simulink model "ELECTRIC_DRIVE"  (R2023a)
settings: Solver=ode1  StartTime=0.0  StopTime=tsim  FixedStep=CONTROL.Tm  RelTol=1e-3
undefined symbols (not defined in the file): CONTROL, MOTOR, myev, SENSOR, speed, tfalta, Tload, Vdc, VSC
libraries: simulink x9
(part 2 of 2)

== matlab function ELECTRIC_DRIVE/TORQUE CONTROL/Variant Subsystem/Vf_5Ph/Vf 5Phase PMSM ==
  settings: updateMethod=DISCRETE
  data: Vphase output; wm input; CONTROL parameter; Vdc parameter
function Vphase  = Vf_5PH(wm, CONTROL, Vdc)

% Variable init
persistent cntr;
persistent wm_km1;
persistent wt_km1;
persistent V_ph;

if isempty(cntr)
    cntr   = CONTROL.N_calc;
    wm_km1 = 0;
    wt_km1 = 0;
    V_ph   = zeros(5,1);
end


%---------  CONTROL LOOP  ---------%
if (cntr==CONTROL.N_calc)
    cntr=0;

    %----- VOLTAGE AMPLITUDE -----%
    Vn     = Vdc/2;
    V = Vn * wm/CONTROL.wm_n;

    %----- INTEGRATOR -----%
    wt = CONTROL.Ts*(wm + wm_km1)/2 + wt_km1;
    wm_km1 = wm;
    wt_km1 = wt;

    %----- VOLTAGE REFERENCE -----%
    ang    = 2*pi/CONTROL.Phase;
    V_ph(1,1) = V * cos(wt);
    V_ph(2,1) = V * cos(wt + ang);
    V_ph(3,1) = V * cos(wt + 2*ang);
    V_ph(4,1) = V * cos(wt + 3*ang);
    V_ph(5,1) = V * cos(wt + 4*ang);

end
cntr = cntr + 1;

%----- ACTUATION -----%
Vphase = V_ph;

end

== matlab function ELECTRIC_DRIVE/MOTOR/Variant Subsystem/PMSM_9Ph/ab2dq1 ==
  data: idq input; iab output; th input
function iab = Park(idq,th)

Mp= [ cos(th)  -sin(th)   0  0  0  0
      sin(th)   cos(th)   0  0  0  0
         0           0    1  0  0  0
         0           0    0  1  0  0
         0           0    0  0  1  0
         0           0    0  0  0  1];

iab = Mp*idq;
end

== matlab function ELECTRIC_DRIVE/TORQUE CONTROL/Variant Subsystem/MPC_9Ph_PMSM/MPC 9Phase PMSM ==
  settings: updateMethod=DISCRETE
  data: Iabc_med input; Sout output; vectores output; Tref input; wm input; th input; Fc_out output; IdqRef output; IabRef output; Iab_km1 output; ch output; CONTROL parameter; SENSOR parameter
function [Sout, vectores, Fc_out, IdqRef, IabRef, Iab_km1, ch] = FCS_MPC_9PH_PMSM(Iabc_med, Tref, wm, th, CONTROL, SENSOR)

% Variable init
persistent uk;
persistent cntr;
persistent x_opt;
% persistent Fc_ana;
persistent Fc;
persistent J_opt;
persistent dq_ref;
persistent Iab_ref;
persistent Sout_km1;
persistent cambios;
persistent Iabxy_med;
persistent Id_med;
persistent Iq_med;
persistent xkp1;
persistent Pkm1;

persistent th_km2;

persistent GAMMA;
persistent GAMMA_Vab;

if isempty(cntr)
    uk  = [0 0 0 0 0]';
    cntr= CONTROL.N_calc;
    Iab_ref = zeros(5,1);
    xkp1 = zeros(5,1);
    dq_ref = zeros(5,1);
    % Fc_ana = zeros(3*length(V_abxy) ,1);
    Fc     = 0;
    Sout_km1 = zeros(length(CONTROL.VECT.S(:,1)),1);
    Sout = zeros(length(CONTROL.VECT.S(:,1)),1);
    cambios = 0;
    x_opt = 0;
    Iabxy_med = zeros(CONTROL.Phase,1);
    Id_med = 0;
    Iq_med = 0;
    Pkm1 = zeros(5,5);

    th_km2 = th;

    GAMMA = CONTROL.B * CONTROL.Ts;
    GAMMA_Vab = GAMMA * CONTROL.Vdc*CONTROL.VECT.V_abxy;
end


%---------  CONTROL LOOP  ---------%
if (cntr==CONTROL.N_calc)
    cntr=0;

    we=wm*CONTROL.P;               % Electric speed
    th_km2 = th + 2*CONTROL.Ts*we; % Orientation correction

    % if MTPA == 1
    %     % v_max =  k_fw*Vdc/2;
    %     Is = sqrt(Id_ref^2 + Iq_ref^2);
    %     kfilt = 0.4;
    %     Iq_med_filt = kfilt*Iq_med + (1-kfilt)*Iq_med_filt;
    %     Id_med_filt = kfilt*Id_med + (1-kfilt)*Id_med_filt;
    % 
    %     Cond_1 = (v_max/we)^2;
    %     Cond_2 = (EMcontrolMPC.Lq*Iq_med_filt)^2+(EMcontrolMPC.Ld*Id_med_filt+EMcontrolMPC.Lambda)^2;
    % 
    %     if 0.8* Cond_1 > Cond_2   % Para evitar singularidades de las referencias de FW
    %         Id_ref = (-EMcontrolMPC.Lambda+sqrt(EMcontrolMPC.Lambda^2 + 8*((EMcontrolMPC.Ld-EMcontrolMPC.Lq)^2)*Is^2)) / (4*(EMcontrolMPC.Ld-EMcontrolMPC.Lq));
    %         Iq_ref = (2*Te_ref) / ( 9*EMcontrolMPC.P * (EMcontrolMPC.Lambda+(EMcontrolMPC.Ld-EMcontrolMPC.Lq)*Id_ref) );
    %     else
    %         Id_ref_mtpa = (-EMcontrolMPC.Lambda+sqrt(EMcontrolMPC.Lambda^2 + 8*((EMcontrolMPC.Ld-EMcontrolMPC.Lq)^2)*Is^2)) / (4*(EMcontrolMPC.Ld-EMcontrolMPC.Lq));
    %         Iq_ref_mtpa = (2*Te_ref) / ( 9*EMcontrolMPC.P * (EMcontrolMPC.Lambda+(EMcontrolMPC.Ld-EMcontrolMPC.Lq)*Id_ref_mtpa) );
    % 
    %         arg = (EMcontrolMPC.Lambda * EMcontrolMPC.Ld)^2 - (EMcontrolMPC.Ld^2 - EMcontrolMPC.Lq^2) * (EMcontrolMPC.Lambda + (EMcontrolMPC.Lq^2) * Is^2 - (v_max^2) / we^2);
    %         if arg > 0 % Control del argumento de la raiz
    %             Id_ref_fw   = (-EMcontrolMPC.Lambda * EMcontrolMPC.Ld + sqrt( arg )) / (EMcontrolMPC.Ld^2 - EMcontrolMPC.Lq^2);
    %             Iq_ref_fw   = (2*Te_ref) / ( 9*EMcontrolMPC.P * (EMcontrolMPC.Lambda+(EMcontrolMPC.Ld-EMcontrolMPC.Lq)*Id_ref_fw) );
    %             beta_mtpa = atan2(Iq_ref_mtpa, Id_ref_mtpa);
    %             beta_fw   = atan2(Iq_ref_fw  , Id_ref_fw  );
    % 
    %             if beta_fw < beta_mtpa   % Zona MTPA
    %                 Id_ref = Id_ref_mtpa;
    %                 Iq_ref = Iq_ref_mtpa;
    % 
    %             else % Zona Field Weakening
    %                 Id_ref = Id_ref_fw;
    %                 Iq_ref = Iq_ref_fw;
    %             end
    %         else
    %             Id_ref = Id_ref_mtpa;
    %             Iq_ref = Iq_ref_mtpa;
    %         end
    %     end
    % else
    % Iq_ref = (2/9)*Te_ref / (EMcontrolMPC.P*EMcontrolMPC.Lambda);
    % end

    %----- REFERENCE CURRENTS -----%
    Id_ref  = 0;
    Iq_ref  = (2/CONTROL.Phase) * Tref/(CONTROL.P*CONTROL.Lambda); 
    Id2_ref = 0;
    Iq2_ref = 0;
    Id3_ref = 0;
    Iq3_ref = 0;
    Ih_ref  = 0;

    % Saturation
    if (Iq_ref >= CONTROL.In)
        Iq_ref = CONTROL.In;
    elseif (Iq_ref <= -CONTROL.In)
        Iq_ref = -CONTROL.In;
    end

    % Inverse Park transform
    Ia_ref = Id_ref*cos(th_km2)    - Iq_ref*sin(th_km2);
    Ib_ref = Id_ref*sin(th_km2)    + Iq_ref*cos(th_km2);
    Ix1_ref = 0; % Id2_ref*cos(3*th_km2) - Iq2_ref*sin(3*th_km2);
    Iy1_ref = 0; % Id2_ref*sin(3*th_km2) + Iq2_ref*cos(3*th_km2);
    Ix2_ref = 0; % Id2_ref*cos(3*th_km2) - Iq2_ref*sin(3*th_km2);
    Iy2_ref = 0; % Id2_ref*sin(3*th_km2) + Iq2_ref*cos(3*th_km2);

    dq_ref  = [Id_ref Iq_ref  Id2_ref Iq2_ref  Id3_ref Iq3_ref  Ih_ref]';
    Iab_ref = [Ia_ref Ib_ref  Ix1_ref Iy1_ref  Ix2_ref Iy2_ref  Ih_ref]';

    %-----   STATE SPACE   -----%
    Ap=[ 0    (CONTROL.Lq*we)/CONTROL.Ld  0    0    0    0
    (CONTROL.Ld*we)/CONTROL.Lq  0         0    0    0    0
         0                      0         0    0    0    0
         0                      0         0    0    0    0
         0                      0         0    0    0    0
         0                      0         0    0    0    0];
    FI=(eye(CONTROL.Phase) + (CONTROL.A+Ap) *CONTROL.Ts); % Discrete state space

    Bemf = [0 -(lambda*we)/Lq 0 0 0 0]';

    %-----  CURRENT MEASUREMENT  -----%
    Iph_sensor = Iabc_med + SENSOR.CURRENT.sigma*randn(9,1);
    
    %  Filtro de Kalman 
    if CONTROL.KALMAN.ACTIVE == 1
        Iph_k = CONTROL.invClarke * xkp1;
        Pk = FI*Pkm1*inv(FI) + CONTROL.KALMAN.Q;
        kk = Pk*inv(Pk + CONTROL.KALMAN.R);
        Iph_filt = Iph_k + kk*(Iph_sensor - Iph_k);
        Pkm1 = (eye(5)-kk)*Pk;
    else
        Iph_filt = Iph_sensor;
    end

    Iabxy_med = CONTROL.Clarke*Iph_filt;
    Id_med =  Iabxy_med(1)*cos(th) + Iabxy_med(2)*sin(th); %Transformada de Park sincrona
    Iq_med = -Iabxy_med(1)*sin(th) + Iabxy_med(2)*cos(th);
    xk = [Id_med Iq_med Iabxy_med(3) Iabxy_med(4) Iabxy_med(5)  Iabxy_med(6) Iabxy_med(7) Iabxy_med(8) Iabxy_med(9)]';

    %----- PREDICTION k+1 -----%
    xkp1=FI*xk + GAMMA*(uk + Bemf);

    %----- PREDICTION k+2 (CONSTANT) -----%
    xkp2_cnst = FI*xkp1 + Bemf*CONTROL.Ts;

    %---- OPTIMIZATION LOOP - PREDICTION k+2 ----%
    Mp= [ cos(th) sin(th) 0  0  0  0 
         -sin(th) cos(th) 0  0  0  0
           0       0      1  0  0  0
           0       0      0  1  0  0
           0       0      0  0  1  0
           0       0      0  0  0  1];

    GAMMA_Vdq = Mp*GAMMA_Vab(1:6,:);
    J_opt = inf; %Inicializacion de la funcion de coste
    for m=1:length(CONTROL.VECT.indx)
        xkp2  = xkp2_cnst + GAMMA_Vdq(:,CONTROL.VECT.indx(m));% xkp2  = FI*xkp1 + GAMMA*V_abxy(:,m) + DELTA;
        error = dq_ref - xkp2;

        Fc1 = error(1)^2 + CONTROL.Kd*error(2)^2;
        Fc2 = CONTROL.Kx1*error(3)^2 + CONTROL.Ky1*error(4)^2;
        Fc3 = CONTROL.Kx2*error(5)^2 + CONTROL.Ky2*error(6)^2;
        %Fc3 = CONTROL.Kh*(error(5)^2);    % Fc_ana(m) = Fc1; Fc_ana(m + length(V_abxy)) = Fc2; Fc_ana(m + 2*length(V_abxy)) = Fc3;

        Fc = Fc1 + Fc2 + Fc3;

        if (Fc < J_opt)
            J_opt=Fc;
            x_opt = m;
        end
    end
    % Voltage vector update
    uk = CONTROL.Vdc* Mp * CONTROL.VECT.V_abxy(:,CONTROL.VECT.indx(x_opt));

    % Swith_km2ing frec. calculation
    cambios = cambios + sum(abs(CONTROL.VECT.S(:,CONTROL.VECT.indx(x_opt)) - Sout_km1)); 
    Sout_km1 = CONTROL.VECT.S(:,CONTROL.VECT.indx(x_opt));
end
cntr = cntr + 1;

%----- ACTUATION -----%
Sout = Sout_km1;

% Output Variable Update
IdqRef = dq_ref;
IabRef = Iab_ref;
Iab_km1 = xkp1;
Fc_out = Fc;
vectores = CONTROL.VECT.indx(x_opt);
ch = cambios;
end

== matlab function ELECTRIC_DRIVE/MOTOR/Variant Subsystem/IM_6Ph/ab2dq ==
  data: Vabxy input; Vdqxy output; th input
 function Vdqxy = Park(Vabxy,th)

% Mp= [ cos(th)   sin(th)           0         0          0
%      -sin(th)   cos(th)           0         0          0 
%          0           0        cos(3*th)   -sin(3*th)   0
%          0           0        sin(3*th)    cos(3*th)   0
%          0           0            0         0          1];
Vdqxy = zeros(5,1);
Mp= [ cos(th)   sin(th)  0  0  0
     -sin(th)   cos(th)  0  0  0 
         0           0   1  0  0
         0           0   0  1  0
         0           0   0  0  1];

Vdqxy = Mp*Vabxy;
end

== matlab function ELECTRIC_DRIVE/TORQUE CONTROL/Variant Subsystem/FOC_5Ph/FOC 5Phase PMSM ==
  settings: updateMethod=DISCRETE
  data: Iabc_med input; Vph_ref output; Tref input; wm input; th input; IdqRef output; IabRef output; CONTROL parameter; SENSOR parameter; VdqRef output; VabRef output
function [Vph_ref, IdqRef, IabRef, VdqRef, VabRef] = FOC_5PH_PMSM(Iabc_med, Tref, wm, th, CONTROL, SENSOR)

% Variable init
persistent cntr;
persistent Vabc_ref;
persistent dq_ref;
persistent Iab_ref;
persistent Iabxy_med;
persistent Vdqxy_ref Vabxy;
persistent Pkm1;

persistent iderror_km1 idinte_km1 iqerror_km1 iqinte_km1;
persistent id3error_km1 id3inte_km1 iq3error_km1 iq3inte_km1 iherror_km1 ihinte_km1;

if isempty(cntr)
    Vabc_ref  = zeros(5,1);%[0 0 0 0 0]';
    cntr= CONTROL.N_calc;
    Iab_ref = zeros(5,1);
    dq_ref = zeros(5,1);
    Iabxy_med = zeros(CONTROL.Phase,1);
    Vdqxy_ref = zeros(5,1); Vabxy = zeros(5,1);
    iderror_km1 = 0; idinte_km1 = 0; iqerror_km1 = 0; iqinte_km1 = 0;
    id3error_km1 = 0; id3inte_km1 = 0; iq3error_km1 = 0; iq3inte_km1 = 0; iherror_km1 = 0; ihinte_km1 = 0;
    Pkm1 = zeros(5,5);
end


%---------  CONTROL LOOP  ---------%
if (cntr==CONTROL.N_calc)
    cntr=0;

    %------- REFERENCE CURRENTS -------%
    Id_ref  = 0;
    Iq_ref  = (2/CONTROL.Phase) * Tref/(CONTROL.P*CONTROL.Lambda); 
    Id3_ref = 0;
    Iq3_ref = 0;
    Ih_ref  = 0;

    % Saturation
    if (Iq_ref >= CONTROL.In)
        Iq_ref = CONTROL.In;
    elseif (Iq_ref <= -CONTROL.In)
        Iq_ref = -CONTROL.In;
    end

    % Inverse Park transform
    Ia_ref = Id_ref*cos(th)    - Iq_ref*sin(th);
    Ib_ref = Id_ref*sin(th)    + Iq_ref*cos(th);
    Ix_ref = Id3_ref*cos(3*th) - Iq3_ref*sin(3*th);
    Iy_ref = Id3_ref*sin(3*th) + Iq3_ref*cos(3*th);

    dq_ref  = [Id_ref Iq_ref Id3_ref Iq3_ref Ih_ref]';
    Iab_ref = [Ia_ref Ib_ref Ix_ref  Iy_ref  Ih_ref]';


    %-------  CURRENT MEASUREMENT  -------%
    % Iph_sensor = Iabc_med + SENSOR.CURRENT.sigma*randn(5,1);
    % 
    % %  Filtro de Kalman 
    % if CONTROL.KALMAN.ACTIVE == 1
    %     Iph_k = CONTROL.invClarke * xkp1;
    %     Pk = FI*Pkm1*inv(FI) + CONTROL.KALMAN.Q;
    %     kk = Pk*inv(Pk + CONTROL.KALMAN.R);
    %     Iph_filt = Iph_k + kk*(Iph_sensor - Iph_k);
    %     Pkm1 = (eye(5)-kk)*Pk;
    % else
    %     Iph_filt = Iph_sensor;
    % end
    Iph_filt = Iabc_med;

    Iabxy_med = CONTROL.Clarke*Iph_filt;

    Id_mea  =  Iabxy_med(1)*cos(th)   + Iabxy_med(2)*sin(th);
    Iq_mea  = -Iabxy_med(1)*sin(th)   + Iabxy_med(2)*cos(th);
    Id3_mea =  Iabxy_med(3)*cos(3*th) + Iabxy_med(4)*sin(3*th); 
    Iq3_mea = -Iabxy_med(3)*sin(3*th) + Iabxy_med(4)*cos(3*th);
    Ih_mea  =  Iabxy_med(5);


    %------------------ PI: D Voltage ------------------%
    id_error=Id_ref-Id_mea; 
    idinte_k = 0.5*CONTROL.Ts*(id_error+iderror_km1)+idinte_km1;
    Vd_ref = CONTROL.id.Kp*id_error + CONTROL.id.Ki*idinte_k;

        % Update variables
        iderror_km1 = id_error;
        idinte_km1  = idinte_k;

    %------------------ PI: Q Voltage ------------------%
    iq_error=Iq_ref-Iq_mea; 
    iqinte_k = 0.5*CONTROL.Ts*(iq_error+iqerror_km1)+iqinte_km1;
    Vq_ref = CONTROL.iq.Kp*iq_error + CONTROL.iq.Ki*iqinte_k;

        % Update variables
        iqerror_km1 = iq_error;
        iqinte_km1  = iqinte_k;

    %------------------ PI: D3 Voltage ------------------%
    id3_error=Id3_ref-Id3_mea; 
    id3inte_k = 0.5*CONTROL.Ts*(id3_error+id3error_km1)+id3inte_km1;
    Vd3_ref = CONTROL.id3.Kp*id3_error + CONTROL.id3.Ki*id3inte_k;

        % Update variables
        id3error_km1 = id3_error;
        id3inte_km1  = id3inte_k;

    %------------------ PI: Q3 Voltage ------------------%
    iq3_error=Iq3_ref-Iq3_mea; 
    iq3inte_k = 0.5*CONTROL.Ts*(iq3_error+iq3error_km1)+iq3inte_km1;
    Vq3_ref = CONTROL.iq3.Kp*iq3_error + CONTROL.iq3.Ki*iq3inte_k;

        % Update variables
        iq3error_km1 = iq3_error;
        iq3inte_km1  = iq3inte_k;

    %------------- PI: zero-sequence Voltage -------------%
    ih_error=Ih_ref-Ih_mea;
    ihinte_k = 0.5*CONTROL.Ts*(ih_error+iherror_km1)+ihinte_km1;
    Vh_ref = CONTROL.ih.Kp*ih_error + CONTROL.ih.Ki*ihinte_k;

        % Update variables
        iherror_km1 = ih_error;
        ihinte_km1  = ihinte_k;


    %-------  REFERENCE VOLTAGE TRANSFORMATIONS  -------%
    Vdqxy_ref = [Vd_ref; Vq_ref; Vd3_ref; Vq3_ref; Vh_ref];

    % Alpha-beta voltage
    Valpha_ref =  Vd_ref*cos(th)  - Vq_ref*sin(th); %Transformada de Park sincrona
    Vbeta_ref  =  Vd_ref*sin(th)  + Vq_ref*cos(th);
    Vx_ref   =  Vd3_ref*cos(3*th) - Vq3_ref*sin(3*th); %Transformada de Park anti-sincrona
    Vy_ref   =  Vd3_ref*sin(3*th) + Vq3_ref*cos(3*th);

    Vabxy = [Valpha_ref; Vbeta_ref; Vx_ref; Vy_ref; Vh_ref];

    % Phase voltage
    Vabc_ref = CONTROL.invClarke*Vabxy;
end
cntr = cntr + 1;

%----- ACTUATION -----%
Vph_ref = Vabc_ref;

% Output Variable Update
IdqRef = dq_ref;
IabRef = Iab_ref;
VdqRef = Vdqxy_ref;
VabRef = Vabxy;
end

== matlab function ELECTRIC_DRIVE/TORQUE CONTROL/Variant Subsystem/FOC_5Ph/MODULATION STAGE/DutyCicle ==
  data: dph input; dl output
function dl = fcn(dph)

dl = zeros(10,1);

if dph(1)>0
    dl(1) = dph(1);
else
    dl(6) = -1*dph(1);
end

if dph(2)>0
    dl(2) = dph(2);
else
    dl(7) = -1*dph(2);
end

if dph(3)>0
    dl(3) = dph(3);
else
    dl(8) = -1*dph(3);
end

if dph(4)>0
    dl(4) = dph(4);
else
    dl(9) = -1*dph(4);
end

if dph(5)>0
    dl(5) = dph(5);
else
    dl(10) = -1*dph(5);
end

== matlab function ELECTRIC_DRIVE/TORQUE CONTROL/Output select ==
  data: o4 input; vect output; o5 input; o6 input; ch output; Iabkm1 output; Vdq_ref output; Vab_ref output; CONTROL parameter
function [vect, ch, Iabkm1, Vdq_ref, Vab_ref]   = output(o4,o5,o6, CONTROL)

vect = 0;
ch = 0;
Iabkm1 = zeros(CONTROL.Phase,1);    
Vdq_ref = zeros(CONTROL.Phase,1);
Vab_ref = zeros(CONTROL.Phase,1);

if CONTROL.Index == 51 || CONTROL.Index == 91  % MPC
    vect = o4;
    ch   = o5;
    Iabkm1 = o6;
elseif CONTROL.Index == 52 || CONTROL.Index == 92 % FOC 
    Vdq_ref = o4;
    Vab_ref = o5;
end

end

== matlab function ELECTRIC_DRIVE/TORQUE CONTROL/Variant Subsystem/FOC_6Ph/FOC 6Phase PMSM ==
  settings: updateMethod=DISCRETE
  data: Iabc_med input; Vph_ref output; Tref input; wm input; th input; IdqRef output; IabRef output; CONTROL parameter; SENSOR parameter; VdqRef output; VabRef output
function [Vph_ref, IdqRef, IabRef, VdqRef, VabRef] = FOC_6PH(Iabc_med, Tref, wm, th, CONTROL, SENSOR)

% Variable init
persistent cntr;
persistent Vabc_ref;
persistent dq_ref;
persistent Iab_ref;
persistent Iabxy_med;
persistent Vdqxy_ref Vabxy;
persistent Pkm1;

persistent iderror_km1 idinte_km1 iqerror_km1 iqinte_km1;
persistent id3error_km1 id3inte_km1 iq3error_km1 iq3inte_km1 iherror_km1 ihinte_km1;

if isempty(cntr)
    Vabc_ref  = zeros(5,1);%[0 0 0 0 0]';
    cntr= CONTROL.N_calc;
    Iab_ref = zeros(5,1);
    dq_ref = zeros(5,1);
    Iabxy_med = zeros(CONTROL.Phase,1);
    Vdqxy_ref = zeros(5,1); Vabxy = zeros(5,1);
    iderror_km1 = 0; idinte_km1 = 0; iqerror_km1 = 0; iqinte_km1 = 0;
    id3error_km1 = 0; id3inte_km1 = 0; iq3error_km1 = 0; iq3inte_km1 = 0; iherror_km1 = 0; ihinte_km1 = 0;
    Pkm1 = zeros(5,5);
end


%---------  CONTROL LOOP  ---------%
if (cntr==CONTROL.N_calc)
    cntr=0;

    %------- REFERENCE CURRENTS -------%
    Id_ref  = 0;
    Iq_ref  = (2/CONTROL.Phase) * Tref/(CONTROL.P*CONTROL.Lambda); 
    Id5_ref = 0;
    Iq5_ref = 0;

    % Saturation
    if (Iq_ref >= CONTROL.In)
        Iq_ref = CONTROL.In;
    elseif (Iq_ref <= -CONTROL.In)
        Iq_ref = -CONTROL.In;
    end

    % Inverse Park transform
    Ia_ref = Id_ref*cos(th)    - Iq_ref*sin(th);
    Ib_ref = Id_ref*sin(th)    + Iq_ref*cos(th);
    Ix_ref = Id3_ref*cos(3*th) - Iq3_ref*sin(3*th);
    Iy_ref = Id3_ref*sin(3*th) + Iq3_ref*cos(3*th);

    dq_ref  = [Id_ref Iq_ref Id3_ref Iq3_ref Ih_ref]';
    Iab_ref = [Ia_ref Ib_ref Ix_ref  Iy_ref  Ih_ref]';


    %-------  CURRENT MEASUREMENT  -------%
    % Iph_sensor = Iabc_med + SENSOR.CURRENT.sigma*randn(5,1);
    % 
    % %  Filtro de Kalman 
    % if CONTROL.KALMAN.ACTIVE == 1
    %     Iph_k = CONTROL.invClarke * xkp1;
    %     Pk = FI*Pkm1*inv(FI) + CONTROL.KALMAN.Q;
    %     kk = Pk*inv(Pk + CONTROL.KALMAN.R);
    %     Iph_filt = Iph_k + kk*(Iph_sensor - Iph_k);
    %     Pkm1 = (eye(5)-kk)*Pk;
    % else
    %     Iph_filt = Iph_sensor;
    % end
    Iph_filt = Iabc_med;

    Iabxy_med = CONTROL.Clarke*Iph_filt;

    Id_mea  =  Iabxy_med(1)*cos(th)   + Iabxy_med(2)*sin(th);
    Iq_mea  = -Iabxy_med(1)*sin(th)   + Iabxy_med(2)*cos(th);
    Id3_mea =  Iabxy_med(3)*cos(3*th) + Iabxy_med(4)*sin(3*th); 
    Iq3_mea = -Iabxy_med(3)*sin(3*th) + Iabxy_med(4)*cos(3*th);
    Ih_mea  =  Iabxy_med(5);


    %------------------ PI: D Voltage ------------------%
    id_error=Id_ref-Id_mea; 
    idinte_k = 0.5*CONTROL.Ts*(id_error+iderror_km1)+idinte_km1;
    Vd_ref = CONTROL.id.Kp*id_error + CONTROL.id.Ki*idinte_k;

        % Update variables
        iderror_km1 = id_error;
        idinte_km1  = idinte_k;

    %------------------ PI: Q Voltage ------------------%
    iq_error=Iq_ref-Iq_mea; 
    iqinte_k = 0.5*CONTROL.Ts*(iq_error+iqerror_km1)+iqinte_km1;
    Vq_ref = CONTROL.iq.Kp*iq_error + CONTROL.iq.Ki*iqinte_k;

        % Update variables
        iqerror_km1 = iq_error;
        iqinte_km1  = iqinte_k;

    %------------------ PI: D3 Voltage ------------------%
    id3_error=Id3_ref-Id3_mea; 
    id3inte_k = 0.5*CONTROL.Ts*(id3_error+id3error_km1)+id3inte_km1;
    Vd3_ref = CONTROL.id3.Kp*id3_error + CONTROL.id3.Ki*id3inte_k;

        % Update variables
        id3error_km1 = id3_error;
        id3inte_km1  = id3inte_k;

    %------------------ PI: Q3 Voltage ------------------%
    iq3_error=Iq3_ref-Iq3_mea; 
    iq3inte_k = 0.5*CONTROL.Ts*(iq3_error+iq3error_km1)+iq3inte_km1;
    Vq3_ref = CONTROL.iq3.Kp*iq3_error + CONTROL.iq3.Ki*iq3inte_k;

        % Update variables
        iq3error_km1 = iq3_error;
        iq3inte_km1  = iq3inte_k;

    %------------- PI: zero-sequence Voltage -------------%
    ih_error=Ih_ref-Ih_mea;
    ihinte_k = 0.5*CONTROL.Ts*(ih_error+iherror_km1)+ihinte_km1;
    Vh_ref = CONTROL.ih.Kp*ih_error + CONTROL.ih.Ki*ihinte_k;

        % Update variables
        iherror_km1 = ih_error;
        ihinte_km1  = ihinte_k;


    %-------  REFERENCE VOLTAGE TRANSFORMATIONS  -------%
    Vdqxy_ref = [Vd_ref; Vq_ref; Vd3_ref; Vq3_ref; Vh_ref];

    % Alpha-beta voltage
    Valpha_ref =  Vd_ref*cos(th)  - Vq_ref*sin(th); %Transformada de Park sincrona
    Vbeta_ref  =  Vd_ref*sin(th)  + Vq_ref*cos(th);
    Vx_ref   =  Vd3_ref*cos(3*th) - Vq3_ref*sin(3*th); %Transformada de Park anti-sincrona
    Vy_ref   =  Vd3_ref*sin(3*th) + Vq3_ref*cos(3*th);

    Vabxy = [Valpha_ref; Vbeta_ref; Vx_ref; Vy_ref; Vh_ref];

    % Phase voltage
    Vabc_ref = CONTROL.invClarke*Vabxy;
end
cntr = cntr + 1;

%----- ACTUATION -----%
Vph_ref = Vabc_ref;

% Output Variable Update
IdqRef = dq_ref;
IabRef = Iab_ref;
VdqRef = Vdqxy_ref;
VabRef = Vabxy;
end

== matlab function ELECTRIC_DRIVE/TORQUE CONTROL/Variant Subsystem/FOC_6Ph/MODULATION STAGE/DutyCicle ==
  data: dph input; dl output
function dl = fcn(dph)

dl = zeros(10,1);

if dph(1)>0
    dl(1) = dph(1);
else
    dl(6) = -1*dph(1);
end

if dph(2)>0
    dl(2) = dph(2);
else
    dl(7) = -1*dph(2);
end

if dph(3)>0
    dl(3) = dph(3);
else
    dl(8) = -1*dph(3);
end

if dph(4)>0
    dl(4) = dph(4);
else
    dl(9) = -1*dph(4);
end

if dph(5)>0
    dl(5) = dph(5);
else
    dl(10) = -1*dph(5);
end

== matlab function ELECTRIC_DRIVE/MOTOR/Variant Subsystem/PMSM_9Ph/ab2dq ==
  data: Vabxy input; Vdqxy output; th input
function Vdqxy = Park(Vabxy,th)

Mp= [ cos(th)   sin(th)   0  0  0  0
     -sin(th)   cos(th)   0  0  0  0
         0           0    1  0  0  0
         0           0    0  1  0  0
         0           0    0  0  1  0
         0           0    0  0  0  1];

Vdqxy = Mp*Vabxy;
end

== matlab function ELECTRIC_DRIVE/TORQUE CONTROL/Variant Subsystem/Hybrid_PI&MPC/Hybrid PIdq and MPCh 5Ph ==
  settings: updateMethod=DISCRETE
  data: Iabc_med input; Vph_ref output; Tref input; wm input; th input; IdqRef output; IabRef output; CONTROL parameter; SENSOR parameter; VdqRef output; VabRef output
function [Vph_ref, IdqRef, IabRef, VdqRef, VabRef] = Hybrid_PIMPC(Iabc_med, Tref, wm, th, CONTROL, SENSOR)

% Variable init
persistent cntr;
persistent Vabc_ref;
persistent dq_ref;
persistent Iab_ref;
persistent Iabxy_med;
persistent Vdqxy_ref Vabxy;
persistent Pkm1;

persistent iderror_km1 idinte_km1 iqerror_km1 iqinte_km1;
persistent id3error_km1 id3inte_km1 iq3error_km1 iq3inte_km1 iherror_km1 ihinte_km1;

persistent FIh GAMMAh uh_k;

if isempty(cntr)
    Vabc_ref  = zeros(5,1);%[0 0 0 0 0]';
    cntr= CONTROL.N_calc;
    Iab_ref = zeros(5,1);
    dq_ref = zeros(5,1);
    Iabxy_med = zeros(CONTROL.Phase,1);
    Vdqxy_ref = zeros(5,1); Vabxy = zeros(5,1);
    iderror_km1 = 0; idinte_km1 = 0; iqerror_km1 = 0; iqinte_km1 = 0;
    id3error_km1 = 0; id3inte_km1 = 0; iq3error_km1 = 0; iq3inte_km1 = 0; iherror_km1 = 0; ihinte_km1 = 0;
    Pkm1 = zeros(5,5);

    uh_k = 0;
    FIh    = (1 + CONTROL.Ah*CONTROL.Ts);
    GAMMAh = CONTROL.Bh * CONTROL.Ts;
end


%---------  CONTROL LOOP  ---------%
if (cntr==CONTROL.N_calc)
    cntr=0;
    we = wm*CONTROL.P;

    %------- REFERENCE CURRENTS -------%
    Id_ref  = 0;
    Iq_ref  = (2/CONTROL.Phase) * Tref/(CONTROL.P*CONTROL.Lambda); 
    Id3_ref = 0;
    Iq3_ref = 0;
    Ih_ref  = 0;

    % Saturation
    if (Iq_ref >= CONTROL.In)
        Iq_ref = CONTROL.In;
    elseif (Iq_ref <= -CONTROL.In)
        Iq_ref = -CONTROL.In;
    end

    % Inverse Park transform
    Ia_ref = Id_ref*cos(th)    - Iq_ref*sin(th);
    Ib_ref = Id_ref*sin(th)    + Iq_ref*cos(th);
    Ix_ref = Id3_ref*cos(3*th) - Iq3_ref*sin(3*th);
    Iy_ref = Id3_ref*sin(3*th) + Iq3_ref*cos(3*th);

    dq_ref  = [Id_ref Iq_ref Id3_ref Iq3_ref Ih_ref]';
    Iab_ref = [Ia_ref Ib_ref Ix_ref  Iy_ref  Ih_ref]';


    %-------  CURRENT MEASUREMENT  -------%
    % Iph_sensor = Iabc_med + SENSOR.CURRENT.sigma*randn(5,1);
    % 
    % %  Filtro de Kalman 
    % if CONTROL.KALMAN.ACTIVE == 1
    %     Iph_k = CONTROL.invClarke * xkp1;
    %     Pk = FI*Pkm1*inv(FI) + CONTROL.KALMAN.Q;
    %     kk = Pk*inv(Pk + CONTROL.KALMAN.R);
    %     Iph_filt = Iph_k + kk*(Iph_sensor - Iph_k);
    %     Pkm1 = (eye(5)-kk)*Pk;
    % else
    %     Iph_filt = Iph_sensor;
    % end
    Iph_filt = Iabc_med;

    Iabxy_med = CONTROL.Clarke*Iph_filt;

    Id_mea  =  Iabxy_med(1)*cos(th)   + Iabxy_med(2)*sin(th);
    Iq_mea  = -Iabxy_med(1)*sin(th)   + Iabxy_med(2)*cos(th);
    Id3_mea =  Iabxy_med(3)*cos(3*th) + Iabxy_med(4)*sin(3*th); 
    Iq3_mea = -Iabxy_med(3)*sin(3*th) + Iabxy_med(4)*cos(3*th);
    Ih_mea  =  Iabxy_med(5);


    %------------------ PI: D Voltage ------------------%
    id_error=Id_ref-Id_mea; 
    idinte_k = 0.5*CONTROL.Ts*(id_error+iderror_km1)+idinte_km1;
    Vd_ref = CONTROL.id.Kp*id_error + CONTROL.id.Ki*idinte_k;

        % Update variables
        iderror_km1 = id_error;
        idinte_km1  = idinte_k;

    %------------------ PI: Q Voltage ------------------%
    iq_error=Iq_ref-Iq_mea; 
    iqinte_k = 0.5*CONTROL.Ts*(iq_error+iqerror_km1)+iqinte_km1;
    Vq_ref = CONTROL.iq.Kp*iq_error + CONTROL.iq.Ki*iqinte_k;

        % Update variables
        iqerror_km1 = iq_error;
        iqinte_km1  = iqinte_k;

    %------------------ PI: D3 Voltage ------------------%
    id3_error=Id3_ref-Id3_mea; 
    id3inte_k = 0.5*CONTROL.Ts*(id3_error+id3error_km1)+id3inte_km1;
    Vd3_ref = CONTROL.id3.Kp*id3_error + CONTROL.id3.Ki*id3inte_k;

        % Update variables
        id3error_km1 = id3_error;
        id3inte_km1  = id3inte_k;

    %------------------ PI: Q3 Voltage ------------------%
    iq3_error=Iq3_ref-Iq3_mea; 
    iq3inte_k = 0.5*CONTROL.Ts*(iq3_error+iq3error_km1)+iq3inte_km1;
    Vq3_ref = CONTROL.iq3.Kp*iq3_error + CONTROL.iq3.Ki*iq3inte_k;

        % Update variables
        iq3error_km1 = iq3_error;
        iq3inte_km1  = iq3inte_k;

    %------------- MPC: zero-sequence Voltage -------------%
    Bemf = we*CONTROL.Eh*sin(5*th);
    ih_kp1 =  FIh*Ih_mea + GAMMAh*(uh_k + Bemf);

    Bemf_km1 = we*CONTROL.Eh*sin(5*(th+we*CONTROL.Ts));
    Vh_ref = inv(GAMMAh) * (-FIh*ih_kp1 + GAMMAh*Bemf_km1);
    % Vh_ref = inv(GAMMAh) * (-FIh*Ih_mea + GAMMAh*Bemf_km1);

    uh_k = Vh_ref;


    %-------  REFERENCE VOLTAGE TRANSFORMATIONS  -------%
    Vdqxy_ref = [Vd_ref; Vq_ref; Vd3_ref; Vq3_ref; Vh_ref];

    % Alpha-beta voltage
    Valpha_ref =  Vd_ref*cos(th)  - Vq_ref*sin(th); %Transformada de Park sincrona
    Vbeta_ref  =  Vd_ref*sin(th)  + Vq_ref*cos(th);
    Vx_ref   =  Vd3_ref*cos(3*th) - Vq3_ref*sin(3*th); %Transformada de Park anti-sincrona
    Vy_ref   =  Vd3_ref*sin(3*th) + Vq3_ref*cos(3*th);

    Vabxy = [Valpha_ref; Vbeta_ref; Vx_ref; Vy_ref; Vh_ref];

    % Phase voltage
    Vabc_ref = CONTROL.invClarke*Vabxy;
end
cntr = cntr + 1;

%----- ACTUATION -----%
Vph_ref = Vabc_ref;

% Output Variable Update
IdqRef = dq_ref;
IabRef = Iab_ref;
VdqRef = Vdqxy_ref;
VabRef = Vabxy;
end

== matlab function ELECTRIC_DRIVE/TORQUE CONTROL/Variant Subsystem/Hybrid_PI&MPC/MODULATION STAGE/DutyCicle ==
  data: dph input; dl output
function dl = fcn(dph)

dl = zeros(10,1);

if dph(1)>0
    dl(1) = dph(1);
else
    dl(6) = -1*dph(1);
end

if dph(2)>0
    dl(2) = dph(2);
else
    dl(7) = -1*dph(2);
end

if dph(3)>0
    dl(3) = dph(3);
else
    dl(8) = -1*dph(3);
end

if dph(4)>0
    dl(4) = dph(4);
else
    dl(9) = -1*dph(4);
end

if dph(5)>0
    dl(5) = dph(5);
else
    dl(10) = -1*dph(5);
end

== matlab function ELECTRIC_DRIVE/SPEED LOOP/SPEED PI CONTROLLER ==
  settings: updateMethod=DISCRETE
  data: T_ref output; wm_ref input; wm input; CONTROL parameter
function T_ref = SPEED_LOOP_PI(wm_ref, wm, CONTROL)

persistent cntr;
persistent e_km1;
persistent inte_km1;
persistent Tref;

if isempty(cntr)
    cntr     = CONTROL.N_calc;
    e_km1    = 0;
    inte_km1 = 0;
    Tref     = 0;
end

%---------  CONTROL LOOP  ---------%
if (cntr==CONTROL.N_calc)
    cntr=0;        

    %-----  SPEED PI  -----%
    werror=wm_ref-wm;                      
    inte_k = 0.5*CONTROL.Ts*(werror+e_km1)+inte_km1;
    Tref = CONTROL.VEL.Kp*(werror+CONTROL.VEL.Ki*inte_k);
    % Update variable
    e_km1=werror;
    inte_km1=inte_k;

end
cntr = cntr + 1;

%----- ACTUATION -----%
T_ref = Tref;

end

== matlab function ELECTRIC_DRIVE/MOTOR/Variant Subsystem/PMSM_5Ph/ab2dq ==
  data: Vabxy input; Vdqxy output; th input
 function Vdqxy = Park(Vabxy,th)

% Mp= [ cos(th)   sin(th)           0         0          0
%      -sin(th)   cos(th)           0         0          0 
%          0           0        cos(3*th)   -sin(3*th)   0
%          0           0        sin(3*th)    cos(3*th)   0
%          0           0            0         0          1];
Vdqxy = zeros(5,1);
Mp= [ cos(th)   sin(th)  0  0  0
     -sin(th)   cos(th)  0  0  0 
         0           0   1  0  0
         0           0   0  1  0
         0           0   0  0  1];

Vdqxy = Mp*Vabxy;
end
